simulink model "afe_rst_inv_psm_distributed_control_two_delays"  (R2026a)
settings: Solver=ode1be  StopTime=simlength  FixedStep=tc  MaxStep=Tc
values from neighbouring files (symbols this model uses):
  Amplitude_U = 1.16    [grid_fault_generator.m]
  Amplitude_V = Amplitude_U    (= 1.16)    [grid_fault_generator.m]
  Amplitude_W = Amplitude_U    (= 1.16)    [grid_fault_generator.m]
  end_time_LVRT = start_time_LVRT + error_length    [grid_fault_generator.m]
  Igrid_phase_normalization_factor = 270*sqrt(2)    [grid_emulator.m]
  omega_grid_emulator_nom = w_grid    (= 314.159265359)    [grid_emulator.m]
  omega_grid_nom = w_grid    (= 314.159265359)    [grid_emulator.m]
  t_ramp = 20e-3    (= 0.02)    [grid_fault_generator.m]
  ugrid_factor = 1    [grid_emulator.m]
  V_phase_normalization_factor = Vgrid_phase_normalization_factor    [grid_emulator.m]
  Vdc_bez = 1070    [grid_emulator.m]
  Vemu_ref_norm = Vemu_ref * sqrt(2) / V_phase_normalization_factor    [grid_emulator.m]
  vn_eta_pu = 0    [grid_emulator.m]
  vn_xi_pu = 0    [grid_emulator.m]
  vp_xi_pu = 1    [grid_emulator.m]
undefined symbols (not defined in the file or in its folder): Adrso, Aresd, Bresd, CFi, CFu, Cresd, Crso, CTRPIFF_CLIP_RELEASE, dead_time_INV, emf_fb_p, emf_fb_p_ccaller_1, emf_fb_p_ccaller_2, emf_p, emf_p_ccaller_1, emf_p_ccaller_2, fPWM_INV, g0_161Hz, g0_500Hz, g1_161Hz, g1_500Hz, i_grid_neg_eta_lim, i_grid_neg_eta_red_lim, i_grid_neg_xi_lim, i_grid_neg_xi_red_lim, i_grid_pos_eta_lim, i_grid_pos_eta_red_lim, ibez, id_lim, ieta_neg_ref_lim, ieta_pos_ref_lim, iq_lim, ixi_pos_ref_lim, Jm_norm, k_frt_ref, kg, ki_afe, ki_i, ki_id, ki_iq, ki_rc_neg_grid, ki_rc_pos_grid, ki_vs, ki_w, kp_afe, kp_i, kp_id, kp_iq, kp_rc_neg_grid, kp_rc_pos_grid, kp_vs, kp_w, kw, l1, l2, Lalpha_norm, Ld_norm, Ldrso, Lq_norm, Ls_norm, luenberger_l1 ... (+30)
libraries: fl_lib x146, nesl_utility x62, simulink x8, cstblocks_lti x7, sl_discontinuities x3, single_phase_transformer_lib x3, flexshaft_lib x1, permanent_magnet_synchronous_machine x1
(part 14 of 14)

== system afe_rst_inv_psm_distributed_control_two_delays/INV-Modular/inv_leg_v/driver_board_v/motor_vector_control/current_ctrl/dq_pi_with_vector_antiwindup/dq_vector_pi/pi_q ==
  iq_tilde : Inport
  clip : Inport  Port=2
  1/Ti : Gain  Gain=kp_iq  SaturateOnIntegerOverflow=on  OutDataTypeStr=Inherit: Same as input  ParamDataTypeStr=Inherit: Same as input
  Constant : Constant  Value=0
  Constant1 : Constant  Value=Ls_norm
  Product : Product  Inputs=3
  Sum2 : Sum  Inputs=+-  SaturateOnIntegerOverflow=on
  Sum4 : Sum  SaturateOnIntegerOverflow=on
  Sum5 : Sum  Inputs=+++  SaturateOnIntegerOverflow=on
  Switch1 : Switch  Threshold=0.5  SaturateOnIntegerOverflow=off  InputSameDT=off
  Switch2 : Switch  Threshold=0.5  SaturateOnIntegerOverflow=off  InputSameDT=off
  Unit Delay1 : UnitDelay  SampleTime=ts_inv
  Unit Delay2 : UnitDelay  SampleTime=ts_inv
  kp1 : Gain  Gain=CTRPIFF_CLIP_RELEASE*ts_inv  SaturateOnIntegerOverflow=on  OutDataTypeStr=Inherit: Same as input  ParamDataTypeStr=Inherit: Same as input
  kp2 : Gain  Gain=ki_iq*ts_inv  SaturateOnIntegerOverflow=on  OutDataTypeStr=Inherit: Same as input  ParamDataTypeStr=Inherit: Same as input
  kp3 : Gain  Gain=0  SaturateOnIntegerOverflow=on  OutDataTypeStr=Inherit: Same as input  ParamDataTypeStr=Inherit: Same as input
  Vqs_out : Outport  VectorParamsAs1DForOutWhenUnconnected=off
  wires:
  Constant/1 -> Switch2/1
  [clip] -> Switch1/2
  [clip] -> Switch2/2
  clip/1 -> Unit Delay1/1
  kp2/1 -> Switch2/3
  Switch2/1 -> Sum4/1
  1/Ti/1 -> Sum5/1
  Unit Delay2/1 -> Sum2/1, kp1/1, Sum4/2
  Sum2/1 -> Switch1/1
  kp1/1 -> Sum2/2
  Sum4/1 -> Sum5/2, Switch1/3
  Switch1/1 -> Unit Delay2/1
  iq_tilde/1 -> 1/Ti/1, kp2/1
  Unit Delay1/1 -> [clip]
  Sum5/1 -> Vqs_out/1
  [omega_pu_hat_flt] -> Product/1
  [id_inverter_pu] -> Product/2
  Constant1/1 -> Product/3
  Product/1 -> kp3/1
  kp3/1 -> Sum5/3

== system afe_rst_inv_psm_distributed_control_two_delays/INV-Modular/inv_leg_v/driver_board_v/motor_vector_control/current_ctrl/dq_pi_with_vector_antiwindup/dq_vector_pi/switch ==
  clip 1 : Inport
  clip 2 : Inport  Port=2
  Constant4 : Constant
  Constant5 : Constant  Value=0
  Sum1 : Sum  SaturateOnIntegerOverflow=on
  Switch : Switch  Threshold=0.5  SaturateOnIntegerOverflow=off  InputSameDT=off
  clip : Outport  VectorParamsAs1DForOutWhenUnconnected=off
  wires:
  Constant5/1 -> Switch/3
  Switch/1 -> clip/1
  Constant4/1 -> Switch/1
  Sum1/1 -> Switch/2
  clip 1/1 -> Sum1/1
  clip 2/1 -> Sum1/2

== system afe_rst_inv_psm_distributed_control_two_delays/INV-Modular/inv_leg_v/driver_board_v/motor_vector_control/current_ctrl/dq_pi_with_vector_antiwindup/dq_vector_pi/vector lenght ==
  md : Inport
  mq : Inport  Port=2
  Math Function : Math  Operator=magnitude^2  SignedPower=on
  Math Function1 : Math  Operator=magnitude^2  SignedPower=on
  Math Function2 : Math  Operator=reciprocal  SignedPower=on
  Sqrt : Sqrt
  Sum5 : Sum  SaturateOnIntegerOverflow=on
  m_1 : Outport  VectorParamsAs1DForOutWhenUnconnected=off
  m : Outport  Port=2  VectorParamsAs1DForOutWhenUnconnected=off
  wires:
  Sqrt/1 -> m/1, Math Function2/1
  mq/1 -> Math Function1/1
  Math Function1/1 -> Sum5/2
  Math Function/1 -> Sum5/1
  Sum5/1 -> Sqrt/1
  Math Function2/1 -> m_1/1
  md/1 -> Math Function/1

== system afe_rst_inv_psm_distributed_control_two_delays/INV-Modular/inv_leg_v/driver_board_v/motor_vector_control/current_ctrl/dq_pi_with_vector_antiwindup/dq_vector_pi_ccaller/Reset ==
  Step : Step  Time=0.05  InitialValue=1  FinalValue=0  SampleTime=0
  en : Outport
  wires:
  Step/1 -> en/1

== system afe_rst_inv_psm_distributed_control_two_delays/INV-Modular/inv_leg_w/driver_board_w/motor_vector_control/current_ctrl/dq_pi_with_vector_antiwindup/dq_vector_pi/bounder1 ==
  md : Inport
  m_1 : Inport  Port=2
  m : Inport  Port=3
  Constant : Constant
  Constant1 : Constant  Value=0
  Divide : Product
  Switch : Switch  Threshold=pwm_out_lim  SaturateOnIntegerOverflow=off  InputSameDT=off
  Switch1 : Switch  Threshold=pwm_out_lim  SaturateOnIntegerOverflow=off  InputSameDT=off
  md_sat : Outport  VectorParamsAs1DForOutWhenUnconnected=off
  clip : Outport  Port=2  VectorParamsAs1DForOutWhenUnconnected=off
  wires:
  md/1 -> Switch1/3, Divide/2
  m_1/1 -> Divide/1
  Divide/1 -> Switch1/1
  Switch1/1 -> md_sat/1
  Switch/1 -> clip/1
  m/1 -> Switch/2, Switch1/2
  Constant/1 -> Switch/1
  Constant1/1 -> Switch/3

== system afe_rst_inv_psm_distributed_control_two_delays/INV-Modular/inv_leg_w/driver_board_w/motor_vector_control/current_ctrl/dq_pi_with_vector_antiwindup/dq_vector_pi/bounder2 ==
  m : Inport
  m_1 : Inport  Port=2
  mq : Inport  Port=3
  Constant : Constant
  Constant1 : Constant  Value=0
  Divide : Product
  Switch : Switch  Threshold=pwm_out_lim  SaturateOnIntegerOverflow=off  InputSameDT=off
  Switch1 : Switch  Threshold=pwm_out_lim  SaturateOnIntegerOverflow=off  InputSameDT=off
  mq_sat : Outport  VectorParamsAs1DForOutWhenUnconnected=off
  clip : Outport  Port=2  VectorParamsAs1DForOutWhenUnconnected=off
  wires:
  Constant1/1 -> Switch/3
  Constant/1 -> Switch/1
  m/1 -> Switch1/2, Switch/2
  Switch/1 -> clip/1
  Switch1/1 -> mq_sat/1
  Divide/1 -> Switch1/1
  m_1/1 -> Divide/1
  mq/1 -> Divide/2, Switch1/3

== system afe_rst_inv_psm_distributed_control_two_delays/INV-Modular/inv_leg_w/driver_board_w/motor_vector_control/current_ctrl/dq_pi_with_vector_antiwindup/dq_vector_pi/pi_d ==
  id_tilde : Inport
  clip : Inport  Port=2
  1/Ti : Gain  Gain=kp_id  SaturateOnIntegerOverflow=on  OutDataTypeStr=Inherit: Same as input  ParamDataTypeStr=Inherit: Same as input
  Constant : Constant  Value=0
  Constant1 : Constant  Value=Ls_norm
  Product : Product  Inputs=3
  Sum2 : Sum  Inputs=+-  SaturateOnIntegerOverflow=on
  Sum4 : Sum  SaturateOnIntegerOverflow=on
  Sum5 : Sum  Inputs=+++  SaturateOnIntegerOverflow=on
  Switch1 : Switch  Threshold=0.5  SaturateOnIntegerOverflow=off  InputSameDT=off
  Switch2 : Switch  Threshold=0.5  SaturateOnIntegerOverflow=off  InputSameDT=off
  Unit Delay1 : UnitDelay  SampleTime=ts_inv
  Unit Delay2 : UnitDelay  SampleTime=ts_inv
  kp1 : Gain  Gain=CTRPIFF_CLIP_RELEASE*ts_inv  SaturateOnIntegerOverflow=on  OutDataTypeStr=Inherit: Same as input  ParamDataTypeStr=Inherit: Same as input
  kp2 : Gain  Gain=ki_id*ts_inv  SaturateOnIntegerOverflow=on  OutDataTypeStr=Inherit: Same as input  ParamDataTypeStr=Inherit: Same as input
  kp3 : Gain  Gain=0  SaturateOnIntegerOverflow=on  OutDataTypeStr=Inherit: Same as input  ParamDataTypeStr=Inherit: Same as input
  ud_out : Outport  VectorParamsAs1DForOutWhenUnconnected=off
  wires:
  id_tilde/1 -> kp2/1, 1/Ti/1
  Switch1/1 -> Unit Delay2/1
  Sum4/1 -> Sum5/2, Switch1/3
  kp1/1 -> Sum2/2
  Sum2/1 -> Switch1/1
  Unit Delay2/1 -> Sum4/2, kp1/1, Sum2/1
  1/Ti/1 -> Sum5/1
  Switch2/1 -> Sum4/1
  kp2/1 -> Switch2/3
  clip/1 -> Unit Delay1/1
  [clip] -> Switch2/2
  [clip] -> Switch1/2
  Constant/1 -> Switch2/1
  Unit Delay1/1 -> [clip]
  Sum5/1 -> ud_out/1
  [iq_inverter_pu] -> Product/2
  [omega_pu_hat_flt] -> Product/1
  kp3/1 -> Sum5/3
  Constant1/1 -> Product/3
  Product/1 -> kp3/1

== system afe_rst_inv_psm_distributed_control_two_delays/INV-Modular/inv_leg_w/driver_board_w/motor_vector_control/current_ctrl/dq_pi_with_vector_antiwindup/dq_vector_pi/pi_q ==
  iq_tilde : Inport
  clip : Inport  Port=2
  1/Ti : Gain  Gain=kp_iq  SaturateOnIntegerOverflow=on  OutDataTypeStr=Inherit: Same as input  ParamDataTypeStr=Inherit: Same as input
  Constant : Constant  Value=0
  Constant1 : Constant  Value=Ls_norm
  Product : Product  Inputs=3
  Sum2 : Sum  Inputs=+-  SaturateOnIntegerOverflow=on
  Sum4 : Sum  SaturateOnIntegerOverflow=on
  Sum5 : Sum  Inputs=+++  SaturateOnIntegerOverflow=on
  Switch1 : Switch  Threshold=0.5  SaturateOnIntegerOverflow=off  InputSameDT=off
  Switch2 : Switch  Threshold=0.5  SaturateOnIntegerOverflow=off  InputSameDT=off
  Unit Delay1 : UnitDelay  SampleTime=ts_inv
  Unit Delay2 : UnitDelay  SampleTime=ts_inv
  kp1 : Gain  Gain=CTRPIFF_CLIP_RELEASE*ts_inv  SaturateOnIntegerOverflow=on  OutDataTypeStr=Inherit: Same as input  ParamDataTypeStr=Inherit: Same as input
  kp2 : Gain  Gain=ki_iq*ts_inv  SaturateOnIntegerOverflow=on  OutDataTypeStr=Inherit: Same as input  ParamDataTypeStr=Inherit: Same as input
  kp3 : Gain  Gain=0  SaturateOnIntegerOverflow=on  OutDataTypeStr=Inherit: Same as input  ParamDataTypeStr=Inherit: Same as input
  Vqs_out : Outport  VectorParamsAs1DForOutWhenUnconnected=off
  wires:
  Constant/1 -> Switch2/1
  [clip] -> Switch1/2
  [clip] -> Switch2/2
  clip/1 -> Unit Delay1/1
  kp2/1 -> Switch2/3
  Switch2/1 -> Sum4/1
  1/Ti/1 -> Sum5/1
  Unit Delay2/1 -> Sum2/1, kp1/1, Sum4/2
  Sum2/1 -> Switch1/1
  kp1/1 -> Sum2/2
  Sum4/1 -> Sum5/2, Switch1/3
  Switch1/1 -> Unit Delay2/1
  iq_tilde/1 -> 1/Ti/1, kp2/1
  Unit Delay1/1 -> [clip]
  Sum5/1 -> Vqs_out/1
  [omega_pu_hat_flt] -> Product/1
  [id_inverter_pu] -> Product/2
  Constant1/1 -> Product/3
  Product/1 -> kp3/1
  kp3/1 -> Sum5/3

== system afe_rst_inv_psm_distributed_control_two_delays/INV-Modular/inv_leg_w/driver_board_w/motor_vector_control/current_ctrl/dq_pi_with_vector_antiwindup/dq_vector_pi/switch ==
  clip 1 : Inport
  clip 2 : Inport  Port=2
  Constant4 : Constant
  Constant5 : Constant  Value=0
  Sum1 : Sum  SaturateOnIntegerOverflow=on
  Switch : Switch  Threshold=0.5  SaturateOnIntegerOverflow=off  InputSameDT=off
  clip : Outport  VectorParamsAs1DForOutWhenUnconnected=off
  wires:
  Constant5/1 -> Switch/3
  Switch/1 -> clip/1
  Constant4/1 -> Switch/1
  Sum1/1 -> Switch/2
  clip 1/1 -> Sum1/1
  clip 2/1 -> Sum1/2

== system afe_rst_inv_psm_distributed_control_two_delays/INV-Modular/inv_leg_w/driver_board_w/motor_vector_control/current_ctrl/dq_pi_with_vector_antiwindup/dq_vector_pi/vector lenght ==
  md : Inport
  mq : Inport  Port=2
  Math Function : Math  Operator=magnitude^2  SignedPower=on
  Math Function1 : Math  Operator=magnitude^2  SignedPower=on
  Math Function2 : Math  Operator=reciprocal  SignedPower=on
  Sqrt : Sqrt
  Sum5 : Sum  SaturateOnIntegerOverflow=on
  m_1 : Outport  VectorParamsAs1DForOutWhenUnconnected=off
  m : Outport  Port=2  VectorParamsAs1DForOutWhenUnconnected=off
  wires:
  Sqrt/1 -> m/1, Math Function2/1
  mq/1 -> Math Function1/1
  Math Function1/1 -> Sum5/2
  Math Function/1 -> Sum5/1
  Sum5/1 -> Sqrt/1
  Math Function2/1 -> m_1/1
  md/1 -> Math Function/1

== system afe_rst_inv_psm_distributed_control_two_delays/INV-Modular/inv_leg_w/driver_board_w/motor_vector_control/current_ctrl/dq_pi_with_vector_antiwindup/dq_vector_pi_ccaller/Reset ==
  Step : Step  Time=0.05  InitialValue=1  FinalValue=0  SampleTime=0
  en : Outport
  wires:
  Step/1 -> en/1

== matlab function afe_rst_inv_psm_distributed_control_two_delays/grid/grid_emulator/grid_emulator/voltage_reference/xieta2alphabeta_pos ==
  data: xi input; alpha output; eta input; gamma input; beta output
function [alpha,beta] = xieta2alphabeta_pos(xi,eta,gamma)

    alpha  =  xi*cos(gamma) - eta*sin(gamma);
    beta = xi*sin(gamma) + eta*cos(gamma);

end

== matlab function afe_rst_inv_psm_distributed_control_two_delays/INV-Modular/inv_leg_v/driver_board_v/double_integrator_observer/bounder1 ==
  data: u input; y output
function y = bounder(u)
    
    u = -pi + mod(u+3*pi,2*pi);
    
    y = u;
end

== matlab function afe_rst_inv_psm_distributed_control_two_delays/INV-Modular/inv_leg_v/driver_board_v/double_integrator_observer/bounder2 ==
  data: u input; y output
function y = bounder(u)
    
    u = -pi + mod(u+3*pi,2*pi);
    
    y = u;
end

== matlab function afe_rst_inv_psm_distributed_control_two_delays/INV-Modular/inv_leg_w/driver_board_w/double_integrator_observer/bounder1 ==
  data: u input; y output
function y = bounder(u)
    
    u = -pi + mod(u+3*pi,2*pi);
    
    y = u;
end

== matlab function afe_rst_inv_psm_distributed_control_two_delays/brake/MATLAB Function ==
  data: u input; y output; udc_ref input
function y = fcn(u,udc_ref)

persistent enable_brake

udc_brake_min = 1.145;
udc_brake_max = 1.165;

if isempty(enable_brake)
    enable_brake = 0
end

if u >= udc_ref*udc_brake_max
    y = 15;
    enable_brake = 1;
elseif (u < udc_ref*udc_brake_max && u >= udc_ref*udc_brake_min && enable_brake == 1)
    y = 15;
    enable_brake = 1;
elseif (u < udc_ref*udc_brake_max && u >= udc_ref*udc_brake_min && enable_brake == 0)
    y = 0;
    enable_brake = 0;
else
    y = 0;
    enable_brake = 0;
end

== matlab function afe_rst_inv_psm_distributed_control_two_delays/INV-Modular/inv_leg_v/driver_board_v/motor_vector_control/current_transformation/alphabeta2dq ==
  data: alpha input; d output; beta input; gamma input; q output
function [d,q] = alphabeta2dq(alpha,beta,gamma)

    d  =  alpha*cos(gamma) + beta*sin(gamma);
    q = -alpha*sin(gamma) + beta*cos(gamma);

end

== matlab function afe_rst_inv_psm_distributed_control_two_delays/AFE-Modular/afe_leg_c/driver_board_c/current_ctrl/phase_current_control/MATLAB Function ==
  data: a input; alpha output; b input; c input; beta output
function [alpha,beta] = abc2alphabeta(a,b,c)

alpha = 2/3*(a - 1/2*b - 1/2*c);
beta  = 1/sqrt(3)*(b - c);

end

== matlab function afe_rst_inv_psm_distributed_control_two_delays/INV-Modular/inv_leg_w/driver_board_w/double_integrator_observer/bounder2 ==
  data: u input; y output
function y = bounder(u)
    
    u = -pi + mod(u+3*pi,2*pi);
    
    y = u;
end

== matlab function afe_rst_inv_psm_distributed_control_two_delays/AFE-Modular/afe_leg_b/driver_board_b/current_ctrl/phase_current_control/MATLAB Function ==
  data: a input; alpha output; b input; c input; beta output
function [alpha,beta] = abc2alphabeta(a,b,c)

alpha = 2/3*(a - 1/2*b - 1/2*c);
beta  = 1/sqrt(3)*(b - c);

end

== matlab function afe_rst_inv_psm_distributed_control_two_delays/AFE-Modular/afe_leg_a/driver_board_a/current_ctrl/xieta2abc/MATLAB Function2 ==
  data: alpha input; a output; beta input; b output; c output
function [a,b,c] = alphabeta2abc(alpha,beta)

a = alpha;
b = -(1/2)*alpha + sqrt(3)/2*beta;
c = -(1/2)*alpha - sqrt(3)/2*beta;

end

== matlab function afe_rst_inv_psm_distributed_control_two_delays/AFE-Modular/afe_leg_a/driver_board_a/current_ctrl/xieta2abc/Negative Sequence ==
  data: xi input; alpha output; eta input; gamma input; beta output
function [alpha,beta] = neg2alphabeta(xi,eta,gamma)

    alpha = xi*cos(gamma)  + eta*sin(gamma);
    beta  = -xi*sin(gamma) + eta*cos(gamma);

end

== matlab function afe_rst_inv_psm_distributed_control_two_delays/AFE-Modular/afe_leg_a/driver_board_a/current_ctrl/xieta2abc/Positive Sequence ==
  data: xi input; alpha output; eta input; gamma input; beta output
function [alpha,beta] = pos2alphabeta(xi,eta,gamma)

    alpha = xi*cos(gamma) - eta*sin(gamma);
    beta  = xi*sin(gamma) + eta*cos(gamma);

end

== matlab function afe_rst_inv_psm_distributed_control_two_delays/AFE-Modular/afe_leg_a/driver_board_a/dq_pll/pll_stageA/sequences/alphabeta2xieta/alphabeta2xieta_pos ==
  data: alpha input; xi output; beta input; gamma input; eta output
function [xi,eta] = alphabeta2xieta_pos(alpha,beta,gamma)

    xi  =  alpha*cos(gamma) + beta*sin(gamma);
    eta = -alpha*sin(gamma) + beta*cos(gamma);

end

== matlab function afe_rst_inv_psm_distributed_control_two_delays/AFE-Modular/afe_leg_a/driver_board_a/dq_pll/pll_stageB/bounder1 ==
  data: u input; y output
function y = bounder(u)
    
    u = -pi + mod(u+3*pi,2*pi);
    
    y = u;
end

== matlab function afe_rst_inv_psm_distributed_control_two_delays/AFE-Modular/afe_leg_b/driver_board_b/current_ctrl/xieta2abc/MATLAB Function2 ==
  data: alpha input; a output; beta input; b output; c output
function [a,b,c] = alphabeta2abc(alpha,beta)

a = alpha;
b = -(1/2)*alpha + sqrt(3)/2*beta;
c = -(1/2)*alpha - sqrt(3)/2*beta;

end

== matlab function afe_rst_inv_psm_distributed_control_two_delays/AFE-Modular/afe_leg_b/driver_board_b/current_ctrl/xieta2abc/Negative Sequence ==
  data: xi input; alpha output; eta input; gamma input; beta output
function [alpha,beta] = neg2alphabeta(xi,eta,gamma)

    alpha = xi*cos(gamma)  + eta*sin(gamma);
    beta  = -xi*sin(gamma) + eta*cos(gamma);

end

== matlab function afe_rst_inv_psm_distributed_control_two_delays/AFE-Modular/afe_leg_b/driver_board_b/current_ctrl/xieta2abc/Positive Sequence ==
  data: xi input; alpha output; eta input; gamma input; beta output
function [alpha,beta] = pos2alphabeta(xi,eta,gamma)

    alpha = xi*cos(gamma) - eta*sin(gamma);
    beta  = xi*sin(gamma) + eta*cos(gamma);

end

== matlab function afe_rst_inv_psm_distributed_control_two_delays/AFE-Modular/afe_leg_c/driver_board_c/current_ctrl/xieta2abc/MATLAB Function2 ==
  data: alpha input; a output; beta input; b output; c output
function [a,b,c] = alphabeta2abc(alpha,beta)

a = alpha;
b = -(1/2)*alpha + sqrt(3)/2*beta;
c = -(1/2)*alpha - sqrt(3)/2*beta;

end

== matlab function afe_rst_inv_psm_distributed_control_two_delays/mainboard_afe/dq_pll/pll_stageA/abc_to_alphabeta/abc2alphabeta ==
  data: a input; alpha output; b input; c input; beta output
function [alpha,beta] = abc2alphabeta(a,b,c)

alpha = 2/3*(a - 1/2*b - 1/2*c);
beta  = 1/sqrt(3)*(b - c);

end

== matlab function afe_rst_inv_psm_distributed_control_two_delays/mainboard_afe/dq_pll/pll_stageA/sequences/alphabeta2xieta/alphabeta2xieta_neg ==
  data: alpha input; xi output; beta input; gamma input; eta output
function [xi,eta] = alphabeta2xieta_neg(alpha,beta,gamma)

    xi  = alpha*cos(gamma) - beta*sin(gamma);
    eta = alpha*sin(gamma) + beta*cos(gamma);

end

== matlab function afe_rst_inv_psm_distributed_control_two_delays/mainboard_afe/dq_pll/pll_stageA/sequences/alphabeta2xieta/alphabeta2xieta_pos ==
  data: alpha input; xi output; beta input; gamma input; eta output
function [xi,eta] = alphabeta2xieta_pos(alpha,beta,gamma)

    xi  =  alpha*cos(gamma) + beta*sin(gamma);
    eta = -alpha*sin(gamma) + beta*cos(gamma);

end

== matlab function afe_rst_inv_psm_distributed_control_two_delays/mainboard_afe/dq_pll/pll_stageB/double_integrator_observer/bounder1 ==
  data: u input; y output
function y = bounder(u)
    
    u = -pi + mod(u+3*pi,2*pi);
    
    y = u;
end

== matlab function afe_rst_inv_psm_distributed_control_two_delays/mainboard_afe/dq_pll/pll_stageB/double_integrator_observer/bounder2 ==
  data: u input; y output
function y = bounder(u)
    
    u = -pi + mod(u+3*pi,2*pi);
    
    y = u;
end

== matlab function afe_rst_inv_psm_distributed_control_two_delays/mainboard_afe/dq_pll/pll_stageB/bounder1 ==
  data: u input; y output
function y = bounder(u)
    
    u = -pi + mod(u+3*pi,2*pi);
    
    y = u;
end

== matlab function afe_rst_inv_psm_distributed_control_two_delays/grid/grid_emulator/grid_emulator/phase_gen/bounder1 ==
  data: u input; y output
function y = bounder(u)
    
    u = -pi + mod(u+3*pi,2*pi);
    
    y = u;
end

== matlab function afe_rst_inv_psm_distributed_control_two_delays/INV-Modular/inv_leg_v/driver_board_v/motor_vector_control/current_transformation/uvw2alphabeta ==
  data: u input; alpha output; v input; w input; beta output
function [alpha,beta] = uvw2alphabeta(u,v,w)

alpha = 2/3*(u - 1/2*v - 1/2*w);
beta  = 2/3*(sqrt(3)/2*(v - w));

end

== matlab function afe_rst_inv_psm_distributed_control_two_delays/AFE-Modular/afe_leg_a/modulator/sv_pwm/alphabeta2uvw ==
  data: alpha input; u output; beta input; v output; w output
function [u,v,w] = alphabeta2uvw(alpha,beta)

u  = alpha;
v  = -0.5*alpha+sqrt(3)/2*beta;
w  = -0.5*alpha-sqrt(3)/2*beta;

end

== matlab function afe_rst_inv_psm_distributed_control_two_delays/AFE-Modular/afe_leg_c/driver_board_c/current_ctrl/xieta2abc/Negative Sequence ==
  data: xi input; alpha output; eta input; gamma input; beta output
function [alpha,beta] = neg2alphabeta(xi,eta,gamma)

    alpha = xi*cos(gamma)  + eta*sin(gamma);
    beta  = -xi*sin(gamma) + eta*cos(gamma);

end

== matlab function afe_rst_inv_psm_distributed_control_two_delays/mainboard_afe/ug_alphabeta2xieta/MATLAB Function ==
  data: alpha input; xi output; beta input; gamma input; eta output
function [xi,eta] = alphabeta2pos(alpha,beta,gamma)

    xi  =  alpha*cos(gamma) + beta*sin(gamma);
    eta = -alpha*sin(gamma) + beta*cos(gamma);

end

== matlab function afe_rst_inv_psm_distributed_control_two_delays/mainboard_afe/ug_alphabeta2xieta/MATLAB Function1 ==
  data: alpha input; xi output; beta input; gamma input; eta output
function [xi,eta] = alphabeta2neg(alpha,beta,gamma)

    xi  = alpha*cos(gamma) - beta*sin(gamma);
    eta = alpha*sin(gamma) + beta*cos(gamma);

end

== matlab function afe_rst_inv_psm_distributed_control_two_delays/mainboard_afe/grid_voltage_sampling_and_alpha_beta_transformation/v_abc2alphabeta ==
  data: v_abc input; alpha output; beta output
function [alpha,beta] = abc2alphabeta(v_abc)

alpha = 2/3*(v_abc(1) - 1/2*v_abc(2) - 1/2*v_abc(3));
beta  = 1/sqrt(3)*(v_abc(2) - v_abc(3));

end

== matlab function afe_rst_inv_psm_distributed_control_two_delays/mainboard_afe/ig_alphabeta2xieta/MATLAB Function ==
  data: alpha input; xi output; beta input; gamma input; eta output
function [xi,eta] = alphabeta2pos(alpha,beta,gamma)

    xi  =  alpha*cos(gamma) + beta*sin(gamma);
    eta = -alpha*sin(gamma) + beta*cos(gamma);

end

== matlab function afe_rst_inv_psm_distributed_control_two_delays/mainboard_afe/ig_alphabeta2xieta/MATLAB Function1 ==
  data: alpha input; xi output; beta input; gamma input; eta output
function [xi,eta] = alphabeta2neg(alpha,beta,gamma)

    xi  = alpha*cos(gamma) - beta*sin(gamma);
    eta = alpha*sin(gamma) + beta*cos(gamma);

end

== matlab function afe_rst_inv_psm_distributed_control_two_delays/mainboard_afe/grid_current_sampling_and_alpha_beta_transformation/i_abc2alphabeta ==
  data: i_abc input; alpha output; beta output
function [alpha,beta] = abc2alphabeta(i_abc)

alpha = 2/3*(i_abc(1) - 1/2*i_abc(2) - 1/2*i_abc(3));
beta  = 1/sqrt(3)*(i_abc(2) - i_abc(3));

end

== matlab function afe_rst_inv_psm_distributed_control_two_delays/AFE-Modular/afe_leg_a/driver_board_a/iga_dba_estimator/quadrature_shift_filter ==
  data: input input; y output
function y  = quadrature_shift_filter(input)

FLTD2Q_B1 = 0.000966531084866133;
FLTD2Q_B2 = 0.000946498544476605;
FLTD2Q_A1 = -1.93814485260962;
FLTD2Q_A2 = 0.939101367424292;

    persistent x1 x2 y1 y2

    if isempty(x1)
        x1=0;
        x2=0;
        y1=0;
        y2=0;
    end


    o = x1 * FLTD2Q_B1 + x2 * FLTD2Q_B2 - y1 * FLTD2Q_A1 - y2 * FLTD2Q_A2;
    x2 = x1;
    x1 = input;
    y2 = y1;
    y1 = o;
	y = o;
end

== matlab function afe_rst_inv_psm_distributed_control_two_delays/AFE-Modular/afe_leg_b/driver_board_b/igb_dbb_estimator/quadrature_shift_filter ==
  data: input input; y output
function y  = quadrature_shift_filter(input)

FLTD2Q_B1 = 0.000966531084866133;
FLTD2Q_B2 = 0.000946498544476605;
FLTD2Q_A1 = -1.93814485260962;
FLTD2Q_A2 = 0.939101367424292;

    persistent x1 x2 y1 y2

    if isempty(x1)
        x1=0;
        x2=0;
        y1=0;
        y2=0;
    end


    o = x1 * FLTD2Q_B1 + x2 * FLTD2Q_B2 - y1 * FLTD2Q_A1 - y2 * FLTD2Q_A2;
    x2 = x1;
    x1 = input;
    y2 = y1;
    y1 = o;
	y = o;
end

== matlab function afe_rst_inv_psm_distributed_control_two_delays/AFE-Modular/afe_leg_b/driver_board_b/dq_pll/pll_stageA/mormalization_and_transformation/abc2alphabeta ==
  data: a input; alpha output; b input; c input; beta output
function [alpha,beta] = abc2alphabeta(a,b,c)

alpha = 2/3*(a - 1/2*b - 1/2*c);
beta  = 1/sqrt(3)*(b - c);

end

== matlab function afe_rst_inv_psm_distributed_control_two_delays/AFE-Modular/afe_leg_b/driver_board_b/dq_pll/pll_stageA/sequences/alphabeta2xieta/alphabeta2xieta_neg ==
  data: alpha input; xi output; beta input; gamma input; eta output
function [xi,eta] = alphabeta2xieta_neg(alpha,beta,gamma)

    xi  = alpha*cos(gamma) - beta*sin(gamma);
    eta = alpha*sin(gamma) + beta*cos(gamma);

end

== matlab function afe_rst_inv_psm_distributed_control_two_delays/INV-Modular/inv_leg_u/driver_board_u/double_integrator_observer/bounder1 ==
  data: u input; y output
function y = bounder(u)
    
    u = -pi + mod(u+3*pi,2*pi);
    
    y = u;
end

== matlab function afe_rst_inv_psm_distributed_control_two_delays/AFE-Modular/afe_leg_c/driver_board_c/current_ctrl/xieta2abc/Positive Sequence ==
  data: xi input; alpha output; eta input; gamma input; beta output
function [alpha,beta] = pos2alphabeta(xi,eta,gamma)

    alpha = xi*cos(gamma) - eta*sin(gamma);
    beta  = xi*sin(gamma) + eta*cos(gamma);

end

== matlab function afe_rst_inv_psm_distributed_control_two_delays/AFE-Modular/afe_leg_b/driver_board_b/dq_pll/pll_stageA/sequences/alphabeta2xieta/alphabeta2xieta_pos ==
  data: alpha input; xi output; beta input; gamma input; eta output
function [xi,eta] = alphabeta2xieta_pos(alpha,beta,gamma)

    xi  =  alpha*cos(gamma) + beta*sin(gamma);
    eta = -alpha*sin(gamma) + beta*cos(gamma);

end

== matlab function afe_rst_inv_psm_distributed_control_two_delays/AFE-Modular/afe_leg_b/driver_board_b/dq_pll/pll_stageB/bounder1 ==
  data: u input; y output
function y = bounder(u)
    
    u = -pi + mod(u+3*pi,2*pi);
    
    y = u;
end

== matlab function afe_rst_inv_psm_distributed_control_two_delays/AFE-Modular/afe_leg_c/driver_board_c/dq_pll/pll_stageA/mormalization_and_transformation/abc2alphabeta ==
  data: a input; alpha output; b input; c input; beta output
function [alpha,beta] = abc2alphabeta(a,b,c)

alpha = 2/3*(a - 1/2*b - 1/2*c);
beta  = 1/sqrt(3)*(b - c);

end

== matlab function afe_rst_inv_psm_distributed_control_two_delays/AFE-Modular/afe_leg_c/driver_board_c/dq_pll/pll_stageA/sequences/alphabeta2xieta/alphabeta2xieta_neg ==
  data: alpha input; xi output; beta input; gamma input; eta output
function [xi,eta] = alphabeta2xieta_neg(alpha,beta,gamma)

    xi  = alpha*cos(gamma) - beta*sin(gamma);
    eta = alpha*sin(gamma) + beta*cos(gamma);

end

== matlab function afe_rst_inv_psm_distributed_control_two_delays/AFE-Modular/afe_leg_c/driver_board_c/dq_pll/pll_stageA/sequences/alphabeta2xieta/alphabeta2xieta_pos ==
  data: alpha input; xi output; beta input; gamma input; eta output
function [xi,eta] = alphabeta2xieta_pos(alpha,beta,gamma)

    xi  =  alpha*cos(gamma) + beta*sin(gamma);
    eta = -alpha*sin(gamma) + beta*cos(gamma);

end

== matlab function afe_rst_inv_psm_distributed_control_two_delays/AFE-Modular/afe_leg_c/driver_board_c/dq_pll/pll_stageB/bounder1 ==
  data: u input; y output
function y = bounder(u)
    
    u = -pi + mod(u+3*pi,2*pi);
    
    y = u;
end

== matlab function afe_rst_inv_psm_distributed_control_two_delays/AFE-Modular/afe_leg_c/driver_board_c/igc_dbc_estimator/quadrature_shift_filter ==
  data: input input; y output
function y  = quadrature_shift_filter(input)

FLTD2Q_B1 = 0.000966531084866133;
FLTD2Q_B2 = 0.000946498544476605;
FLTD2Q_A1 = -1.93814485260962;
FLTD2Q_A2 = 0.939101367424292;

    persistent x1 x2 y1 y2

    if isempty(x1)
        x1=0;
        x2=0;
        y1=0;
        y2=0;
    end


    o = x1 * FLTD2Q_B1 + x2 * FLTD2Q_B2 - y1 * FLTD2Q_A1 - y2 * FLTD2Q_A2;
    x2 = x1;
    x1 = input;
    y2 = y1;
    y1 = o;
	y = o;
end

== matlab function afe_rst_inv_psm_distributed_control_two_delays/grid/grid_emulator/grid_emulator/voltage_reference/alphabeta2abc ==
  data: alpha input; a output; beta input; b output; c output
function [a,b,c] = alphabeta2abc(alpha,beta)

    a  =  alpha;
    b  =  -0.5*alpha + sqrt(3)/2*beta;
    c  =  -0.5*alpha - sqrt(3)/2*beta;
end

== matlab function afe_rst_inv_psm_distributed_control_two_delays/INV-Modular/inv_leg_u/driver_board_u/motor_vector_control/current_transformation/alphabeta2dq ==
  data: alpha input; d output; beta input; gamma input; q output
function [d,q] = alphabeta2dq(alpha,beta,gamma)

    d  =  alpha*cos(gamma) + beta*sin(gamma);
    q = -alpha*sin(gamma) + beta*cos(gamma);

end

== matlab function afe_rst_inv_psm_distributed_control_two_delays/INV-Modular/inv_leg_u/driver_board_u/motor_vector_control/current_transformation/uvw2alphabeta ==
  data: u input; alpha output; v input; w input; beta output
function [alpha,beta] = uvw2alphabeta(u,v,w)

alpha = 2/3*(u - 1/2*v - 1/2*w);
beta  = 2/3*(sqrt(3)/2*(v - w));

end

== matlab function afe_rst_inv_psm_distributed_control_two_delays/INV-Modular/inv_leg_u/driver_board_u/motor_vector_control/dq2alphabeta ==
  data: d input; alpha output; q input; gamma input; beta output
function [alpha,beta] = dq2alphabeta(d,q,gamma)

    alpha  =  d*cos(gamma) - q*sin(gamma);
    beta = d*sin(gamma) + q*cos(gamma);

end

== matlab function afe_rst_inv_psm_distributed_control_two_delays/INV-Modular/inv_leg_v/driver_board_v/motor_vector_control/dq2alphabeta ==
  data: d input; alpha output; q input; gamma input; beta output
function [alpha,beta] = dq2alphabeta(d,q,gamma)

    alpha  =  d*cos(gamma) - q*sin(gamma);
    beta = d*sin(gamma) + q*cos(gamma);

end

== matlab function afe_rst_inv_psm_distributed_control_two_delays/mainboard_inverter/double_integrator_observer/bounder1 ==
  data: u input; y output
function y = bounder(u)
    
    u = -pi + mod(u+3*pi,2*pi);
    
    y = u;
end

== matlab function afe_rst_inv_psm_distributed_control_two_delays/INV-Modular/inv_leg_w/driver_board_w/motor_vector_control/current_transformation/alphabeta2dq ==
  data: alpha input; d output; beta input; gamma input; q output
function [d,q] = alphabeta2dq(alpha,beta,gamma)

    d  =  alpha*cos(gamma) + beta*sin(gamma);
    q = -alpha*sin(gamma) + beta*cos(gamma);

end

== matlab function afe_rst_inv_psm_distributed_control_two_delays/INV-Modular/inv_leg_w/driver_board_w/motor_vector_control/current_transformation/uvw2alphabeta ==
  data: u input; alpha output; v input; w input; beta output
function [alpha,beta] = uvw2alphabeta(u,v,w)

alpha = 2/3*(u - 1/2*v - 1/2*w);
beta  = 2/3*(sqrt(3)/2*(v - w));

end

== matlab function afe_rst_inv_psm_distributed_control_two_delays/INV-Modular/inv_leg_w/driver_board_w/motor_vector_control/dq2alphabeta ==
  data: d input; alpha output; q input; gamma input; beta output
function [alpha,beta] = dq2alphabeta(d,q,gamma)

    alpha  =  d*cos(gamma) - q*sin(gamma);
    beta = d*sin(gamma) + q*cos(gamma);

end

== matlab function afe_rst_inv_psm_distributed_control_two_delays/mainboard_inverter/double_integrator_observer/bounder2 ==
  data: u input; y output
function y = bounder(u)
    
    u = -pi + mod(u+3*pi,2*pi);
    
    y = u;
end

== matlab function afe_rst_inv_psm_distributed_control_two_delays/INV-Modular/inv_leg_u/modulator/sv_pwm/alphabeta2uvw ==
  data: alpha input; u output; beta input; v output; w output
function [u,v,w] = alphabeta2uvw(alpha,beta)

u  = alpha;
v  = -0.5*alpha+sqrt(3)/2*beta;
w  = -0.5*alpha-sqrt(3)/2*beta;

end

== matlab function afe_rst_inv_psm_distributed_control_two_delays/FRT-VDE4110/FRT-Detection/LVRT_detector ==
  data: vxi_p input; vxi_n input; veta_n input; vxi_p_dot input; vxi_n_dot input; enable input; red_dyn_enabled input; pwr_lim_enable output; frt_exceeded output; reset input; frt_active output; frt_state output; red_dyn_active output
function [pwr_lim_enable, frt_exceeded, frt_active, frt_state, red_dyn_active]  = lvrt_detector(vxi_p,vxi_n,veta_n,vxi_p_dot,vxi_n_dot, enable, red_dyn_enabled, reset)

    persistent state count count2 state_pwr_lim
    
    LVRT_IDLE = 0;
    LVRT_ACTIVE = 1;
    LVRT_EXCEEDED = 2;
    
    PWR_LIM_DISABLED = 0;
    PWR_LIM_ENABLED  = 1;
    
    LVRT_VPOS_TH_LOW			= 0.91;
    LVRT_VPOS_TH_HIGH			= 1.1;
    LVRT_SEQ_DETECTION_HYST		= 0.06;
    LVRT_VNEG_TH				= 0.06;
    LVRT_VPOS_DOT_TH			= 3.0;
    LVRT_VNEG_DOT_TH			= 3.0;
    LVRT_VPOS_PWRLIM_TH			= 0.8;
    LVRT_VNEG_PWRLIM_TH			= 0.06;
    LVRT_PWRLIM_HYST			= 0.05;
    LVRT_VPOS_RED_DYN_TH        = 0.7;
    LVRT_VNEG_RED_DYN_TH        = 0.2;
    LVRT_TIME_HOLD_MAX          = 61000;
    
    RED_DYN_NOT_ACTIVE = 0;
    RED_DYN_ACTIVE     = 1;
        
    if isempty(state)
        state = LVRT_IDLE;
        state_pwr_lim = PWR_LIM_DISABLED;
        count = 0;
        count2 = 0;
    end

    vn = sqrt(vxi_n^2+veta_n^2);

    if enable == 1
        
        switch state
            
            case LVRT_IDLE
                if ((vxi_p > LVRT_VPOS_TH_HIGH || vxi_p < LVRT_VPOS_TH_LOW || vn > LVRT_VNEG_TH) ...
                     && (vxi_p_dot > LVRT_VPOS_DOT_TH || vxi_n_dot > LVRT_VNEG_DOT_TH) && ...
                     count2 > 4000)
                    state = LVRT_ACTIVE;
                end
                frt_active = 0;
                frt_exceeded = 0;
                count = 0;
                frt_state = LVRT_IDLE;
                state_pwr_lim = PWR_LIM_DISABLED;                  
                red_dyn_active = RED_DYN_NOT_ACTIVE;
                count2 = count2 + 1;

            case LVRT_ACTIVE
                count2 = 0;
                % LVRT condition not active anymore
                if (vxi_p >= LVRT_VPOS_TH_LOW  + LVRT_SEQ_DETECTION_HYST && ...
                    vxi_p <  LVRT_VPOS_TH_HIGH - LVRT_SEQ_DETECTION_HYST)
                    state = LVRT_IDLE;
                % LVRT exceeded
                elseif (count >= LVRT_TIME_HOLD_MAX)
                    state = LVRT_EXCEEDED;
                end
                
                % handle power limitation
                if (vxi_p < LVRT_VPOS_PWRLIM_TH || vn > LVRT_VNEG_PWRLIM_TH) 
                    state_pwr_lim = PWR_LIM_ENABLED;
                elseif (vxi_p > LVRT_VPOS_PWRLIM_TH + LVRT_PWRLIM_HYST && vn < LVRT_VPOS_PWRLIM_TH - LVRT_PWRLIM_HYST)
                    state_pwr_lim = PWR_LIM_DISABLED;                  
                end
                
                % handle reduced dynamic grid support
                if red_dyn_enabled && (vxi_p < LVRT_VPOS_RED_DYN_TH || vn > LVRT_VNEG_RED_DYN_TH)
                    red_dyn_active = RED_DYN_ACTIVE;
                else
                    red_dyn_active = RED_DYN_NOT_ACTIVE;
                end
                 
                frt_active = 1;
                frt_exceeded = 0;
                frt_state = LVRT_ACTIVE;
                
                count = count + 1;
            
            case LVRT_EXCEEDED

                if ((reset == 1) || (enable == 0))
                    state = LVRT_IDLE;
                else
                    state = LVRT_EXCEEDED;
                end
                
                frt_exceeded = 1;
                frt_active = 0; 
                frt_state = LVRT_EXCEEDED;
                red_dyn_active = RED_DYN_NOT_ACTIVE;
            
            otherwise
                state = LVRT_IDLE;
                frt_active = 0;
                frt_exceeded = 0;
                frt_state = LVRT_IDLE;
                red_dyn_active = RED_DYN_NOT_ACTIVE;
        end
        
        if state_pwr_lim == PWR_LIM_ENABLED
            pwr_lim_enable = 1;
        else
            pwr_lim_enable = 0;
        end      
    else
        state = LVRT_IDLE;
        frt_active = 0;
        pwr_lim_enable = 0;
        frt_exceeded = 0;
        frt_state = LVRT_IDLE;
        red_dyn_active = RED_DYN_NOT_ACTIVE;
    end
end

== matlab function afe_rst_inv_psm_distributed_control_two_delays/grid/grid_emulator/grid_emulator/voltage_reference/xieta2alphabeta_neg ==
  data: xi input; alpha output; eta input; gamma input; beta output
function [alpha,beta] = xieta2alphabeta_neg(xi,eta,gamma)

    alpha  =  xi*cos(gamma) + eta*sin(gamma);
    beta = -xi*sin(gamma) + eta*cos(gamma);

end

== matlab function afe_rst_inv_psm_distributed_control_two_delays/FRT-VDE4110/FRT-PosNegReactiveCurrentReferences/avg_flt_500ms/avg_flt_1 ==
  data: x input; y1 output; w input; Tc input; enable input
function y1  = avg_flt(x,w,Tc, enable)

    persistent x_int x_int_1 y_N N

    N = (1/(w/(2*pi)))/Tc+1;

    if isempty(x_int)
        x_int_1 = 0;
        y_N = zeros(1,N);
        y1 = 0;
    end


    if enable == 1
        x_int = x * Tc * w + x_int_1;
        x_int_1 = x_int;
        y_N(1,1) = x_int;
        y1 = 1/(2*pi)*((y_N(1,1) - y_N(1,N)));
        for i = 1:(N-1)
            y_N(1,N+1-i) = y_N(1,N-i); 
        end
    else
        y1 = 1/(2*pi)*((y_N(1,1) - y_N(1,N)));
    end
end

== matlab function afe_rst_inv_psm_distributed_control_two_delays/FRT-VDE4110/FRT-PosNegReactiveCurrentReferences/avg_flt_500ms1/avg_flt_1 ==
  data: x input; y1 output; w input; Tc input; enable input
function y1  = avg_flt(x,w,Tc, enable)

    persistent x_int x_int_1 y_N N

    N = (1/(w/(2*pi)))/Tc+1;

    if isempty(x_int)
        x_int_1 = 0;
        y_N = zeros(1,N);
        y1 = 0;
    end


    if enable == 1
        x_int = x * Tc * w + x_int_1;
        x_int_1 = x_int;
        y_N(1,1) = x_int;
        y1 = 1/(2*pi)*((y_N(1,1) - y_N(1,N)));
        for i = 1:(N-1)
            y_N(1,N+1-i) = y_N(1,N-i); 
        end
    else
        y1 = 1/(2*pi)*((y_N(1,1) - y_N(1,N)));
    end
end

== matlab function afe_rst_inv_psm_distributed_control_two_delays/FRT-VDE4110/FRT-PosNegReactiveCurrentReferences/avg_flt_500ms2/avg_flt_1 ==
  data: x input; y1 output; w input; Tc input; enable input
function y1  = avg_flt(x,w,Tc, enable)

    persistent x_int x_int_1 y_N N

    N = (1/(w/(2*pi)))/Tc+1;

    if isempty(x_int)
        x_int_1 = 0;
        y_N = zeros(1,N);
        y1 = 0;
    end


    if enable == 1
        x_int = x * Tc * w + x_int_1;
        x_int_1 = x_int;
        y_N(1,1) = x_int;
        y1 = 1/(2*pi)*((y_N(1,1) - y_N(1,N)));
        for i = 1:(N-1)
            y_N(1,N+1-i) = y_N(1,N-i); 
        end
    else
        y1 = 1/(2*pi)*((y_N(1,1) - y_N(1,N)));
    end
end

== matlab function afe_rst_inv_psm_distributed_control_two_delays/FRT-VDE4110/FRT-PosNegReactiveCurrentReferences/avg_flt_500ms3/avg_flt_1 ==
  data: x input; y1 output; w input; Tc input; enable input
function y1  = avg_flt(x,w,Tc, enable)

    persistent x_int x_int_1 y_N N

    N = (1/(w/(2*pi)))/Tc+1;

    if isempty(x_int)
        x_int_1 = 0;
        y_N = zeros(1,N);
        y1 = 0;
    end


    if enable == 1
        x_int = x * Tc * w + x_int_1;
        x_int_1 = x_int;
        y_N(1,1) = x_int;
        y1 = 1/(2*pi)*((y_N(1,1) - y_N(1,N)));
        for i = 1:(N-1)
            y_N(1,N+1-i) = y_N(1,N-i); 
        end
    else
        y1 = 1/(2*pi)*((y_N(1,1) - y_N(1,N)));
    end
end

== matlab function afe_rst_inv_psm_distributed_control_two_delays/grid/grid_emulator/grid_emulator/voltage_reference/Grid: Voltage-Source in abc/Phase_a1 ==
  data: A input; y output; phi input
function y = Phase_a(A,phi)

    y = A*cos(phi);

end

== matlab function afe_rst_inv_psm_distributed_control_two_delays/grid/grid_emulator/grid_emulator/voltage_reference/Grid: Voltage-Source in abc/Phase_b1 ==
  data: A input; y output; phi input
function y = Phase_b(A,phi)

    y = A*cos(phi-2*pi/3);

end

== matlab function afe_rst_inv_psm_distributed_control_two_delays/grid/grid_emulator/grid_emulator/voltage_reference/Grid: Voltage-Source in abc/Phase_c1 ==
  data: A input; y output; phi input
function y = Phase_c(A,phi)

    y = A*cos(phi-4*pi/3);

end

== matlab function afe_rst_inv_psm_distributed_control_two_delays/INV-Modular/inv_leg_u/driver_board_u/motor_vector_control/bemf_observer/bemf_observer_simulink/double_integrator_observer/bounder1 ==
  data: u input; y output
function y = bounder(u)
    
    u = -pi + mod(u+3*pi,2*pi);
    
    y = u;
end

== matlab function afe_rst_inv_psm_distributed_control_two_delays/INV-Modular/inv_leg_u/driver_board_u/motor_vector_control/bemf_observer/bemf_observer_simulink/double_integrator_observer/bounder2 ==
  data: u input; y output
function y = bounder(u)
    
    u = -pi + mod(u+3*pi,2*pi);
    
    y = u;
end

== matlab function afe_rst_inv_psm_distributed_control_two_delays/INV-Modular/inv_leg_w/driver_board_w/motor_vector_control/bemf_observer/bemf_observer_simulink/double_integrator_observer/bounder1 ==
  data: u input; y output
function y = bounder(u)
    
    u = -pi + mod(u+3*pi,2*pi);
    
    y = u;
end

== matlab function afe_rst_inv_psm_distributed_control_two_delays/INV-Modular/inv_leg_w/driver_board_w/motor_vector_control/bemf_observer/bemf_observer_simulink/double_integrator_observer/bounder2 ==
  data: u input; y output
function y = bounder(u)
    
    u = -pi + mod(u+3*pi,2*pi);
    
    y = u;
end

== matlab function afe_rst_inv_psm_distributed_control_two_delays/AFE-Modular/afe_leg_a/driver_board_a/current_ctrl/phase_current_control/MATLAB Function ==
  data: a input; alpha output; b input; c input; beta output
function [alpha,beta] = abc2alphabeta(a,b,c)

alpha = 2/3*(a - 1/2*b - 1/2*c);
beta  = 1/sqrt(3)*(b - c);

end

== matlab function afe_rst_inv_psm_distributed_control_two_delays/INV-Modular/inv_leg_v/driver_board_v/motor_vector_control/bemf_observer/bemf_observer_simulink/double_integrator_observer/bounder1 ==
  data: u input; y output
function y = bounder(u)
    
    u = -pi + mod(u+3*pi,2*pi);
    
    y = u;
end

== matlab function afe_rst_inv_psm_distributed_control_two_delays/INV-Modular/inv_leg_v/driver_board_v/motor_vector_control/bemf_observer/bemf_observer_simulink/double_integrator_observer/bounder2 ==
  data: u input; y output
function y = bounder(u)
    
    u = -pi + mod(u+3*pi,2*pi);
    
    y = u;
end

== matlab function afe_rst_inv_psm_distributed_control_two_delays/INV-Modular/inv_leg_u/driver_board_u/double_integrator_observer/bounder2 ==
  data: u input; y output
function y = bounder(u)
    
    u = -pi + mod(u+3*pi,2*pi);
    
    y = u;
end

== matlab function afe_rst_inv_psm_distributed_control_two_delays/AFE-Modular/afe_leg_a/driver_board_a/dq_pll/pll_stageA/transformation/abc2alphabeta ==
  data: a input; alpha output; b input; c input; beta output
function [alpha,beta] = abc2alphabeta(a,b,c)

alpha = 2/3*(a - 1/2*b - 1/2*c);
beta  = 1/sqrt(3)*(b - c);

end

== matlab function afe_rst_inv_psm_distributed_control_two_delays/AFE-Modular/afe_leg_a/driver_board_a/dq_pll/pll_stageA/sequences/alphabeta2xieta/alphabeta2xieta_neg ==
  data: alpha input; xi output; beta input; gamma input; eta output
function [xi,eta] = alphabeta2xieta_neg(alpha,beta,gamma)

    xi  = alpha*cos(gamma) - beta*sin(gamma);
    eta = alpha*sin(gamma) + beta*cos(gamma);

end
